simulink model "ASM_Traffic_new"  (R2024a)
settings: Solver=ode1  StartTime=SIM.tstart.v  StopTime=SIM.tend.v  FixedStep=SIM.StepSize.v  RelTol=1e-3
PostLoadFcn:
  | if any(exist('dsrtsu_mdlpostloadfcn', 'file') ~= 0), dsrtsu_mdlpostloadfcn('Execute', bdroot); end
  | try, asm_mdl_postloadfcn(bdroot, 'UpdateModel', 3600); catch, disp(lasterr); end,
InitFcn:
  | , if any(exist('rtifpga_mdlclblib', 'file') ~= 0), rtifpga_mdlclblib('Init', bdroot); end,
  | , if any(exist('dsmpb_private', 'file') ~= 0), dsmpb_private('dsmpb_mdlclblib', 'Init', bdroot); end,
undefined symbols (not defined in the file): _to_, a0b2, ASM_BrakeHydraulics_DemoSystems, ASM_VehicleDynamics_DemoSystems, b98103fe8ad365046cd0, BrakeCircuit, CPT, Crankshaft, DiscIntNeverNeededParam, dsmsi, FinalDriveAssembly, MDL, ModeSignals, Pos_BrakePedal_Maneuver, rad, RefSignals, s_to_rpm, SIM, SoftECU, Suspension, Tire, Transmission
libraries: ASM_Traffic_lib x135, simulink x100, ASM_Utils_lib x77, ASM_VehicleDynamics_lib x70, ASM_Environment_lib x22, dsmpblib x20, dsmsilib x15, MDLD_Utils_lib x10, ASM_BrakeHydraulics_lib x3
(part 30 of 63)

== system ASM_Traffic_new/VehicleDynamics/Interface_Out/Plant_ModelSignals/Sw_r_Tire[1:intern;2:extern]_ ==
  In1 : Inport
  Gain : Gain  SaturateOnIntegerOverflow=on  OutDataTypeStr=Inherit: Same as input  ParamDataTypeStr=Inherit: Same as input
  Out1 : Outport  VectorParamsAs1DForOutWhenUnconnected=off
  wires:
  In1/1 -> Gain/1
  Gain/1 -> Out1/1

== system ASM_Traffic_new/VehicleDynamics/Interface_Out/Plant_ModelSignals/Trq_Max_Brake[Nm]_ ==
  In1 : Inport
  Gain : Gain  SaturateOnIntegerOverflow=on  OutDataTypeStr=Inherit: Same as input  ParamDataTypeStr=Inherit: Same as input
  Out1 : Outport  VectorParamsAs1DForOutWhenUnconnected=off
  wires:
  Gain/1 -> Out1/1
  In1/1 -> Gain/1

== system ASM_Traffic_new/VehicleDynamics/Interface_Out/Plant_ModelSignals/Trq_SteeringWheel[Nm]_ ==
  In1 : Inport
  Gain : Gain  SaturateOnIntegerOverflow=on  OutDataTypeStr=Inherit: Same as input  ParamDataTypeStr=Inherit: Same as input
  Out1 : Outport  VectorParamsAs1DForOutWhenUnconnected=off
  wires:
  Gain/1 -> Out1/1
  In1/1 -> Gain/1

== system ASM_Traffic_new/VehicleDynamics/Interface_Out/Plant_ModelSignals/YawRate_Vehicle_CoG[deg|s]_ ==
  In1 : Inport
  Gain : Gain  SaturateOnIntegerOverflow=on  OutDataTypeStr=Inherit: Same as input  ParamDataTypeStr=Inherit: Same as input
  Out1 : Outport  VectorParamsAs1DForOutWhenUnconnected=off
  wires:
  Gain/1 -> Out1/1
  In1/1 -> Gain/1

== system ASM_Traffic_new/VehicleDynamics/Interface_Out/Plant_ModelSignals/a_Vehicle[x;y;z][m|s2]_ ==
  In1 : Inport
  Gain : Gain  SaturateOnIntegerOverflow=on  OutDataTypeStr=Inherit: Same as input  ParamDataTypeStr=Inherit: Same as input
  Out1 : Outport  VectorParamsAs1DForOutWhenUnconnected=off
  wires:
  In1/1 -> Gain/1
  Gain/1 -> Out1/1

== system ASM_Traffic_new/VehicleDynamics/Interface_Out/Plant_ModelSignals/a_x_Vehicle_CoG[m|s2]_ ==
  In1 : Inport
  Gain : Gain  SaturateOnIntegerOverflow=on  OutDataTypeStr=Inherit: Same as input  ParamDataTypeStr=Inherit: Same as input
  Out1 : Outport  VectorParamsAs1DForOutWhenUnconnected=off
  wires:
  Gain/1 -> Out1/1
  In1/1 -> Gain/1

== system ASM_Traffic_new/VehicleDynamics/Interface_Out/Plant_ModelSignals/a_y_Vehicle_CoG[m|s2]_ ==
  In1 : Inport
  Gain : Gain  SaturateOnIntegerOverflow=on  OutDataTypeStr=Inherit: Same as input  ParamDataTypeStr=Inherit: Same as input
  Out1 : Outport  VectorParamsAs1DForOutWhenUnconnected=off
  wires:
  Gain/1 -> Out1/1
  In1/1 -> Gain/1

== system ASM_Traffic_new/VehicleDynamics/Interface_Out/Plant_ModelSignals/a_z_Vehicle_CoG[m|s2]_ ==
  In1 : Inport
  Gain : Gain  SaturateOnIntegerOverflow=on  OutDataTypeStr=Inherit: Same as input  ParamDataTypeStr=Inherit: Same as input
  Out1 : Outport  VectorParamsAs1DForOutWhenUnconnected=off
  wires:
  Gain/1 -> Out1/1
  In1/1 -> Gain/1

== system ASM_Traffic_new/VehicleDynamics/Interface_Out/Plant_ModelSignals/i_Steering_Mean[]_ ==
  In1 : Inport
  Gain : Gain  SaturateOnIntegerOverflow=on  OutDataTypeStr=Inherit: Same as input  ParamDataTypeStr=Inherit: Same as input
  Out1 : Outport  VectorParamsAs1DForOutWhenUnconnected=off
  wires:
  Gain/1 -> Out1/1
  In1/1 -> Gain/1

== system ASM_Traffic_new/VehicleDynamics/Interface_Out/Plant_ModelSignals/m_TotalVehicle[kg]_ ==
  In1 : Inport
  Gain : Gain  SaturateOnIntegerOverflow=on  OutDataTypeStr=Inherit: Same as input  ParamDataTypeStr=Inherit: Same as input
  Out1 : Outport  VectorParamsAs1DForOutWhenUnconnected=off
  wires:
  Gain/1 -> Out1/1
  In1/1 -> Gain/1

== system ASM_Traffic_new/VehicleDynamics/Interface_Out/Plant_ModelSignals/omega_Mean_Wheel[rad|s]_ ==
  In1 : Inport
  Gain : Gain  SaturateOnIntegerOverflow=on  OutDataTypeStr=Inherit: Same as input  ParamDataTypeStr=Inherit: Same as input
  Out1 : Outport  VectorParamsAs1DForOutWhenUnconnected=off
  wires:
  Gain/1 -> Out1/1
  In1/1 -> Gain/1

== system ASM_Traffic_new/VehicleDynamics/Interface_Out/Plant_ModelSignals/omega_Wheel[FL;FR;RL;RR][rad|s]_ ==
  In1 : Inport
  Gain : Gain  SaturateOnIntegerOverflow=on  OutDataTypeStr=Inherit: Same as input  ParamDataTypeStr=Inherit: Same as input
  Out1 : Outport  VectorParamsAs1DForOutWhenUnconnected=off
  wires:
  Gain/1 -> Out1/1
  In1/1 -> Gain/1

== system ASM_Traffic_new/VehicleDynamics/Interface_Out/Plant_ModelSignals/omega_Wheel[rad|s]_ ==
  In1 : Inport
  Gain : Gain  SaturateOnIntegerOverflow=on  OutDataTypeStr=Inherit: Same as input  ParamDataTypeStr=Inherit: Same as input
  Out1 : Outport  VectorParamsAs1DForOutWhenUnconnected=off
  wires:
  Gain/1 -> Out1/1
  In1/1 -> Gain/1

== system ASM_Traffic_new/VehicleDynamics/Interface_Out/Plant_ModelSignals/r_Dyn_Tire[FL;FR;RL;RR][m]_ ==
  In1 : Inport
  Gain : Gain  SaturateOnIntegerOverflow=on  OutDataTypeStr=Inherit: Same as input  ParamDataTypeStr=Inherit: Same as input
  Out1 : Outport  VectorParamsAs1DForOutWhenUnconnected=off
  wires:
  Gain/1 -> Out1/1
  In1/1 -> Gain/1

== system ASM_Traffic_new/VehicleDynamics/Interface_Out/Plant_ModelSignals/r_Tire_extern[m]_ ==
  In1 : Inport
  Gain : Gain  SaturateOnIntegerOverflow=on  OutDataTypeStr=Inherit: Same as input  ParamDataTypeStr=Inherit: Same as input
  Out1 : Outport  VectorParamsAs1DForOutWhenUnconnected=off
  wires:
  In1/1 -> Gain/1
  Gain/1 -> Out1/1

== system ASM_Traffic_new/VehicleDynamics/Interface_Out/Plant_ModelSignals/s_Vehicle[m]_ ==
  In1 : Inport
  Gain : Gain  SaturateOnIntegerOverflow=on  OutDataTypeStr=Inherit: Same as input  ParamDataTypeStr=Inherit: Same as input
  Out1 : Outport  VectorParamsAs1DForOutWhenUnconnected=off
  wires:
  Gain/1 -> Out1/1
  In1/1 -> Gain/1

== system ASM_Traffic_new/VehicleDynamics/Interface_Out/Plant_ModelSignals/v_Vehicle[km|h]_ ==
  In1 : Inport
  Gain : Gain  SaturateOnIntegerOverflow=on  OutDataTypeStr=Inherit: Same as input  ParamDataTypeStr=Inherit: Same as input
  Out1 : Outport  VectorParamsAs1DForOutWhenUnconnected=off
  wires:
  Gain/1 -> Out1/1
  In1/1 -> Gain/1

== system ASM_Traffic_new/VehicleDynamics/Interface_Out/Plant_ModelSignals/v_Vehicle[x;y;z][km|h]_ ==
  In1 : Inport
  Gain : Gain  SaturateOnIntegerOverflow=on  OutDataTypeStr=Inherit: Same as input  ParamDataTypeStr=Inherit: Same as input
  Out1 : Outport  VectorParamsAs1DForOutWhenUnconnected=off
  wires:
  Gain/1 -> Out1/1
  In1/1 -> Gain/1

== system ASM_Traffic_new/VehicleDynamics/Interface_Out/Plant_ModelSignals/v_Vehicle_dt[x;y;z][m|s2]_ ==
  In1 : Inport
  Gain : Gain  SaturateOnIntegerOverflow=on  OutDataTypeStr=Inherit: Same as input  ParamDataTypeStr=Inherit: Same as input
  Out1 : Outport  VectorParamsAs1DForOutWhenUnconnected=off
  wires:
  Gain/1 -> Out1/1
  In1/1 -> Gain/1

== system ASM_Traffic_new/VehicleDynamics/Interface_Out/Plant_ModelSignals/v_x_Vehicle_CoG[km|h]_ ==
  In1 : Inport
  Gain : Gain  SaturateOnIntegerOverflow=on  OutDataTypeStr=Inherit: Same as input  ParamDataTypeStr=Inherit: Same as input
  Out1 : Outport  VectorParamsAs1DForOutWhenUnconnected=off
  wires:
  Gain/1 -> Out1/1
  In1/1 -> Gain/1

== system ASM_Traffic_new/VehicleDynamics/Interface_Out/Plant_ModelSignals/v_y_Vehicle_CoG[km|h]_ ==
  In1 : Inport
  Gain : Gain  SaturateOnIntegerOverflow=on  OutDataTypeStr=Inherit: Same as input  ParamDataTypeStr=Inherit: Same as input
  Out1 : Outport  VectorParamsAs1DForOutWhenUnconnected=off
  wires:
  Gain/1 -> Out1/1
  In1/1 -> Gain/1

== system ASM_Traffic_new/VehicleDynamics/Interface_Out/Plant_ModelSignals/v_z_Vehicle_CoG[km|h]_ ==
  In1 : Inport
  Gain : Gain  SaturateOnIntegerOverflow=on  OutDataTypeStr=Inherit: Same as input  ParamDataTypeStr=Inherit: Same as input
  Out1 : Outport  VectorParamsAs1DForOutWhenUnconnected=off
  wires:
  Gain/1 -> Out1/1
  In1/1 -> Gain/1

== system ASM_Traffic_new/VehicleDynamics/Interface_Out/Plant_ModelSignals/w_Vehicle[x;y;z][deg|s]_ ==
  In1 : Inport
  Gain : Gain  SaturateOnIntegerOverflow=on  OutDataTypeStr=Inherit: Same as input  ParamDataTypeStr=Inherit: Same as input
  Out1 : Outport  VectorParamsAs1DForOutWhenUnconnected=off
  wires:
  Gain/1 -> Out1/1
  In1/1 -> Gain/1

== system ASM_Traffic_new/VehicleDynamics/Interface_Out/Plant_ModelSignals/w_Vehicle_dt[x;y;z][rad|s2]_ ==
  In1 : Inport
  Gain : Gain  SaturateOnIntegerOverflow=on  OutDataTypeStr=Inherit: Same as input  ParamDataTypeStr=Inherit: Same as input
  Out1 : Outport  VectorParamsAs1DForOutWhenUnconnected=off
  wires:
  Gain/1 -> Out1/1
  In1/1 -> Gain/1

== system ASM_Traffic_new/VehicleDynamics/Interface_Out/Plant_ModelSignals/w_x_Vehicle_CoG[rad|s2]_ ==
  In1 : Inport
  Gain : Gain  SaturateOnIntegerOverflow=on  OutDataTypeStr=Inherit: Same as input  ParamDataTypeStr=Inherit: Same as input
  Out1 : Outport  VectorParamsAs1DForOutWhenUnconnected=off
  wires:
  Gain/1 -> Out1/1
  In1/1 -> Gain/1

== system ASM_Traffic_new/VehicleDynamics/Interface_Out/Plant_ModelSignals/w_y_Vehicle_CoG[rad|s2]_ ==
  In1 : Inport
  Gain : Gain  SaturateOnIntegerOverflow=on  OutDataTypeStr=Inherit: Same as input  ParamDataTypeStr=Inherit: Same as input
  Out1 : Outport  VectorParamsAs1DForOutWhenUnconnected=off
  wires:
  In1/1 -> Gain/1
  Gain/1 -> Out1/1

== system ASM_Traffic_new/VehicleDynamics/Interface_Out/Plant_ModelSignals/w_z_Vehicle_CoG[rad|s2]_ ==
  In1 : Inport
  Gain : Gain  SaturateOnIntegerOverflow=on  OutDataTypeStr=Inherit: Same as input  ParamDataTypeStr=Inherit: Same as input
  Out1 : Outport  VectorParamsAs1DForOutWhenUnconnected=off
  wires:
  Gain/1 -> Out1/1
  In1/1 -> Gain/1

== system ASM_Traffic_new/VehicleDynamics/Plant/Sw_Plant_Signals/Angle_Gamma_FL_Wheel[deg] ==
  SoftECU : Inport
  RealECU : Inport  Port=2
  Const_Angle_Gamma_FL_Wheel[deg] : Constant  Value=0
  MultiPortSwitch : MultiPortSwitch
  Sw_Angle_Gamma_FL_Wheel[1SoftECU|2RealECU|3Const] : Constant  Value=CPT.MDL_SW.Sw_Angle_Gamma_FL_Wheel.v
  Angle_Gamma_FL_Wheel[deg] : Outport  VectorParamsAs1DForOutWhenUnconnected=off
  wires:
  MultiPortSwitch/1 -> Angle_Gamma_FL_Wheel[deg]/1
  Const_Angle_Gamma_FL_Wheel[deg]/1 -> MultiPortSwitch/4
  RealECU/1 -> MultiPortSwitch/3
  SoftECU/1 -> MultiPortSwitch/2
  Sw_Angle_Gamma_FL_Wheel[1SoftECU|2RealECU|3Const]/1 -> MultiPortSwitch/1

== system ASM_Traffic_new/VehicleDynamics/Plant/Sw_Plant_Signals/Displ_SteeringRod[Displ;Displ_dt][m;m|s] ==
  SoftECU : Inport
  RealECU : Inport  Port=2
  Const_Displ_SteeringRod[Displ;Displ_dt][m;m|s] : Constant  Value=[0;0]
  MultiPortSwitch : MultiPortSwitch
  Sw_Displ_SteeringRod[1SoftECU|2RealECU|3Const] : Constant  Value=CPT.MDL_SW.Sw_Displ_SteeringRod.v
  Displ_SteeringRod[Displ;Displ_dt][m;m|s] : Outport  VectorParamsAs1DForOutWhenUnconnected=off
  wires:
  MultiPortSwitch/1 -> Displ_SteeringRod[Displ;Displ_dt][m;m|s]/1
  Const_Displ_SteeringRod[Displ;Displ_dt][m;m|s]/1 -> MultiPortSwitch/4
  RealECU/1 -> MultiPortSwitch/3
  SoftECU/1 -> MultiPortSwitch/2
  Sw_Displ_SteeringRod[1SoftECU|2RealECU|3Const]/1 -> MultiPortSwitch/1

== system ASM_Traffic_new/VehicleDynamics/Plant/Sw_Plant_Signals/EPSMotorStates_External[Angle;Angle_dt][rad;rad|s] ==
  SoftECU : Inport
  RealECU : Inport  Port=2
  Const_EPSMotorStates_External[Angle;Angle_dt][rad;rad|s] : Constant  Value=[0;0]
  MultiPortSwitch : MultiPortSwitch
  Sw_EPSMotorStates_External[1SoftECU|2RealECU|3Const] : Constant  Value=CPT.MDL_SW.Sw_EPSMotorStates_External.v
  EPSMotorStates_External[Angle;Angle_dt][rad;rad|s] : Outport  VectorParamsAs1DForOutWhenUnconnected=off
  wires:
  Sw_EPSMotorStates_External[1SoftECU|2RealECU|3Const]/1 -> MultiPortSwitch/1
  SoftECU/1 -> MultiPortSwitch/2
  RealECU/1 -> MultiPortSwitch/3
  Const_EPSMotorStates_External[Angle;Angle_dt][rad;rad|s]/1 -> MultiPortSwitch/4
  MultiPortSwitch/1 -> EPSMotorStates_External[Angle;Angle_dt][rad;rad|s]/1

== system ASM_Traffic_new/VehicleDynamics/Plant/Sw_Plant_Signals/omega_Wheel[FL;FR;RL;RR][rad|s] ==
  SoftECU : Inport
  RealECU : Inport  Port=2
  Const_omega_Wheel[FL;FR;RL;RR][rad|s] : Constant  Value=[0 0 0 0]
  MultiPortSwitch : MultiPortSwitch
  Sw_omega_Wheel[1SoftECU|2RealECU|3Const] : Constant  Value=CPT.MDL_SW.Sw_omega_Wheel.v
  omega_Wheel[FL;FR;RL;RR][rad|s] : Outport  VectorParamsAs1DForOutWhenUnconnected=off
  wires:
  Sw_omega_Wheel[1SoftECU|2RealECU|3Const]/1 -> MultiPortSwitch/1
  SoftECU/1 -> MultiPortSwitch/2
  RealECU/1 -> MultiPortSwitch/3
  MultiPortSwitch/1 -> omega_Wheel[FL;FR;RL;RR][rad|s]/1
  Const_omega_Wheel[FL;FR;RL;RR][rad|s]/1 -> MultiPortSwitch/4

== system ASM_Traffic_new/VehicleDynamics/Plant/UserInterface/ASMSignalBus_Plant ==
  In : Inport
  Terminator_1 : Terminator
  tag scope: ASMBUS_VehicleDynamics_Plant=global
  wires:
  In/1 -> [ASMBUS_VehicleDynamics_Plant]  "Plant"
  [ASMBUS_VehicleDynamics_Plant] -> Terminator_1/1

== system ASM_Traffic_new/VehicleDynamics/Plant/UserInterface/DISP_Plant ==
  In : Inport
  Accelerations : Subsystem
  Aerodynamics : Subsystem
  Brake : Subsystem
  Bus Selector2 : BusSelector  OutputSignals=Suspension,VehicleMovement.Positions,VehicleMovement.Velocities,VehicleMovement.Accelerations,Wheel,Tire,Aerodynamics,Steering,Brake,VehicleMovement.SensorMotion.Sensor1
  Overview : Subsystem
  Positions : Subsystem
  Sensor1 : Subsystem
  Steering : Subsystem
  Suspension : Subsystem
  Tire : Subsystem
  Velocities : Subsystem
  WheelSpeeds : Subsystem
  wires:
  Bus Selector2/10 -> Sensor1/1(Sensor1)  "<Sensor1>"
  Bus Selector2/5 -> WheelSpeeds/1(WheelSpeeds)  "<Wheel>"
  Bus Selector2/4 -> Accelerations/1(Accelerations), Overview/2(Accelerations)  "<Accelerations>"
  In/1 -> Bus Selector2/1
  Bus Selector2/8 -> Steering/1(Steering)  "<Steering>"
  Bus Selector2/3 -> Velocities/1(Velocities), Overview/1(Velocities)  "<Velocities>"
  Bus Selector2/6 -> Tire/1(Tire)  "<Tire>"
  Bus Selector2/7 -> Aerodynamics/1(Aerodynamics)  "<Aerodynamics>"
  Bus Selector2/9 -> Brake/1(Brake)  "<Brake>"
  Bus Selector2/2 -> Positions/1(Positions)  "<Positions>"
  Bus Selector2/1 -> Suspension/1(Suspension)  "<Suspension>"

== system ASM_Traffic_new/VehicleDynamics/Plant/UserInterface/PAR_Plant ==
  BrakeHydraulics_DistributionPattern_Switch : Subsystem
      mask Display: disp('BrakeHydraulics_DistributionPattern_Switch')
  Bus Creator : BusCreator  Inputs=3
  Bus Creator1 : BusCreator  Inputs=1
  Bus Creator2 : BusCreator  Inputs=1
  Bus Creator3 : BusCreator  Inputs=2
  ModelDesk_MC_ID_VehicleDynamics : ASM_Utils_lib/ModelDeskInterface/ModelDesk_MC  Tag=ASM_MAINCOMPONENT  Editable=off  MainComponent=VehicleDynamics
  ROTATION_SWITCH : ASM_VehicleDynamics_lib/VehicleDynamics/Suspension/Common/ROTATION_SWITCH  Tag=ASM_SUBCOMPONENT  Sw_Rotation=MDL.VehicleDynamics.SW_Rotation  ASMProperties=struct('Name','ROTATION_SWITCH','Version','2.0','Library','ASM_VehicleDynamics_lib')  ASMInstanceName=rotation_switch  ASMInstanceID=1
  Suspension_Inits : Subsystem
      mask Display: disp('Suspension Inits')
  Tire_Switches : Subsystem
      mask Display: disp('Tire Switches')
  Out : Outport  VectorParamsAs1DForOutWhenUnconnected=off
  wires:
  ROTATION_SWITCH/1 -> Bus Creator3/2  "Sw_Rotation[1Cardan|2ToeCamberCaster]"
  Bus Creator3/1 -> Bus Creator/3  "Suspension"
  Bus Creator/1 -> Out/1  "UserInterface"
  Bus Creator2/1 -> Bus Creator/2  "BrakeHydraulics"
  Tire_Switches/1(Tire_Switches) -> Bus Creator1/1  "Tire"
  Suspension_Inits/1(Suspension_Init) -> Bus Creator3/1
  BrakeHydraulics_DistributionPattern_Switch/1(Sw_DistributionPattern_[1X|2II]) -> Bus Creator2/1
  Bus Creator1/1 -> Bus Creator/1  "Tire"

== system ASM_Traffic_new/VehicleDynamics/Plant/VehicleDynamics/ASMSignalCollector ==
  Bus Selector : BusSelector  OutputSignals=Coef_RollingRes_Mean[]
  Bus Selector1 : BusSelector  OutputSignals=Forces.F_x_Aero_CoorSys_V[N]
  Bus Selector2 : BusSelector  OutputSignals=MassForcesAndTorques.GravitationalForces.F_Vehicle_Gravitational[x;y;z][N]
  BusCreator : BusCreator  Inputs=9
  Driving_Resistances : Subsystem
  ASMSignalBus : Outport  VectorParamsAs1DForOutWhenUnconnected=off
  wires:
  [ASMBUS_VehicleDynamics_WheelSpeed] -> BusCreator/4
  [ASMBUS_VehicleDynamics_Aerodynamics] -> Bus Selector1/1, BusCreator/3
  [ASMBUS_VehicleDynamics_Brake] -> BusCreator/6
  Driving_Resistances/1(F_Driving_Res[N]) -> BusCreator/9
  Bus Selector2/1 -> Driving_Resistances/1(F_Vehicle_Gravitational[x;y;z][N])  "<F_Vehicle_Gravitational[x;y;z][N]>"
  Bus Selector/1 -> Driving_Resistances/2(Coef_RollingRes_Mean[])  "<Coef_RollingRes_Mean[]>"
  [ASMBUS_VehicleDynamics_Steering] -> BusCreator/5
  [ASMBUS_VehicleDynamics_VehicleMovement] -> Bus Selector2/1, BusCreator/1
  Bus Selector1/1 -> Driving_Resistances/3(F_x_Aero_CoorSys_V[N])  "<F_x_Aero_CoorSys_V[N]>"
  [ASMBUS_VehicleDynamics_Suspension] -> BusCreator/7
  [ASMBUS_VehicleDynamics_Tire] -> Bus Selector/1, BusCreator/2
  BusCreator/1 -> ASMSignalBus/1  "VehicleDynamics"
  [ASMBUS_VehicleDynamics_Steering_Rod_Back_Calc] -> BusCreator/8

== system ASM_Traffic_new/VehicleDynamics/Plant/VehicleDynamics/Brake ==
  Reset[] : Inport
  Pos_BrakePedal[%] : Inport  Port=2
  IO_Signals : Inport  Port=3
  p_Ambient[Pa] : Inport  Port=4
  Sw_ParkingBrake[0Off|1On] : Inport  Port=5
  T_Ambient[degC] : Inport  Port=6
  Pos_AccPedal[%] : Inport  Port=7
  Sw_DistributionPattern[1X|2II] : Inport  Port=8
  ASMSignalCollector : Subsystem
  BRAKE_DISC : ASM_VehicleDynamics_lib/VehicleDynamics/Brake/BRAKE_DISC  Tag=ASM_SUBCOMPONENT  Const_Fric_Coef_FL=MDL.VehicleDynamics.BrakeDisc.FL.Const_Coef_Fric  Const_Fric_Coef_FR=MDL.VehicleDynamics.BrakeDisc.FR.Const_Coef_Fric  Const_Fric_Coef_RL=MDL.VehicleDynamics.BrakeDisc.RL.Const_Coef_Fric  Const_Fric_Coef_RR=MDL.VehicleDynamics.BrakeDisc.RR.Const_Coef_Fric  Const_A_FL=MDL.VehicleDynamics.BrakeDisc.FL.Const_A_Fric  Const_A_FR=MDL.VehicleDynamics.BrakeDisc.FR.Const_A_Fric  Const_A_RL=MDL.VehicleDynamics.BrakeDisc.RL.Const_A_Fric  Const_A_RR=MDL.VehicleDynamics.BrakeDisc.RR.Const_A_Fric  Const_r_FL=MDL.VehicleDynamics.BrakeDisc.FL.Const_r  Const_r_FR=MDL.VehicleDynamics.BrakeDisc.FR.Const_r  Const_r_RL=MDL.VehicleDynamics.BrakeDisc.RL.Const_r  Const_r_RR=MDL.VehicleDynamics.BrakeDisc.RR.Const_r  ASMProperties=struct('Name','BRAKE_DISC','Version','5.0','Library','ASM_VehicleDynamics_lib')  ASMInstanceName=brake_disc  ASMInstanceID=1
  BRAKE_HYDRAULICS : Subsystem  Tag=BrakeHydraulics_BrakeCircuit
  Bus Selector : BusSelector  OutputSignals=Ctrl_HydPump[0_1],Ctrl_PreChargeValve_1[0_1],Ctrl_PreChargeValve_2[0_1],Ctrl_ChangeOverValve_1[0_1],Ctrl_ChangeOverValve_2[0_1],Ctrl_InletValve_FL[0_1],Ctrl_InletValve_FR[0_1],Ctrl_InletValve_RL[0_1],Ctrl_InletValve_RR[0_1],Ctrl_OutletValve_FL[0_1],Ctrl_OutletValve_FR[0_1],Ctrl_OutletValve_RL[0_1],Ctrl_OutletValve_RR[0_1],ECU_ESP_Mode[0None|1ABS|2ESP|3ASR]
  Bus Selector1 : BusSelector  OutputSignals=Enable_p_Brake_Desired[0|1],p_Brake_Desired[bar]
  Constant : Constant  Value=0
  ForceParkingBrake : Subsystem
  Goto Tag Visibility : GotoTagVisibility  GotoTag=TAG_DISP_BrkHyd_MasterBrakeCylinder
  Goto Tag Visibility1 : GotoTagVisibility  GotoTag=ASMBUS_VehicleDynamics_VacuumServo
  Goto Tag Visibility2 : GotoTagVisibility  GotoTag=ASMBUS_VehicleDynamics_Manifold
  Goto Tag Visibility3 : GotoTagVisibility  GotoTag=ASMBUS_VehicleDynamics_BrakeHydraulics
  Goto Tag Visibility4 : GotoTagVisibility  GotoTag=ASMBUS_VehicleDynamics_BrakeDisc
  MANIFOLD_PRESSURE : ASM_VehicleDynamics_lib/VehicleDynamics/Brake/MANIFOLD_PRESSURE  Tag=ASM_SUBCOMPONENT  Map_p_Man=MDL.VehicleDynamics.ManifoldPressure.Map_p_Man  ASMProperties=struct('Name','MANIFOLD_PRESSURE','Version','2.0','Library','ASM_VehicleDynamics_lib')  ASMInstanceName=manifold_pressure  ASMInstanceID=1
  MASTER_BRAKE_CYLINDER : ASM_BrakeHydraulics_lib/BrakeHydraulics/BrakeCylinders/MASTER_BRAKE_CYLINDER  Tag=ASM_SUBCOMPONENT  Const_p_max=MDL.BrkHyd.MasterBrakeCylinderLinear.Const_p_max  Map_BrakeForce=MDL.BrkHyd.MasterBrakeCylinder.Map_BrakeForce  Const_r_piston=MDL.BrkHyd.MasterBrakeCylinder.Const_r_piston  Const_displ_max_piston=MDL.BrkHyd.MasterBrakeCylinder.Const_displ_max_piston  SW_MasterBrakeCylinder_Mode=MDL.BrkHyd.SW_MasterBrakeCylinderType.v  ASMProperties=struct('Name','MASTER_BRAKE_CYLINDER','Version','8.0','Library','ASM_BrakeHydraulics_lib')  ASMInstanceName=master_brake_cylinder  ASMInstanceID=1
  OpenBrakeCircuit : ASM_Utils_lib/Miscellaneous/OpenSystem  popupLibBlk=<select here>  popupTargetDemo=<select here>  Demosystem=BrakeHydraulics_BrakeCircuit  variantLib=ASM_BrakeHydraulics_DemoSystems/BrakeCircuit
  UnitConversion : ASM_Utils_lib/UnitConversion/UnitConversion  Selection=Pa_to_bar
  VACUUM_SERVO : ASM_VehicleDynamics_lib/VehicleDynamics/Brake/VACUUM_SERVO  Tag=ASM_SUBCOMPONENT  Const_F_OutputPoint=MDL.VehicleDynamics.VacuumServo.Const_F_OutputPoint  Const_p_OutputPoint=MDL.VehicleDynamics.VacuumServo.Const_p_OutputPoint  Const_F_Max_PistonRod=MDL.VehicleDynamics.VacuumServo.Const_F_Max_PistonRod  Const_p_nom_VaccumChamber=MDL.VehicleDynamics.VacuumServo.Const_p_nom_VaccumChamber  Const_V_VacuumChamber=MDL.VehicleDynamics.VacuumServo.Const_V_VacuumChamber  Const_V_RearChamber=MDL.VehicleDynamics.VacuumServo.Const_V_RearChamber  Const_A_Connect_BellValve=MDL.VehicleDynamics.VacuumServo.Const_A_Connect_BellValve  Const_A_Boost_BellValve=MDL.VehicleDynamics.VacuumServo.Const_A_Boost_BellValve  Const_A_MainfoldValve=MDL.VehicleDynamics.VacuumServo.Const_A_MainfoldValve  Const_A_Leakage_MainfoldValve=MDL.VehicleDynamics.VacuumServo.Const_A_Leakage_MainfoldValve  Const_c_spring=MDL.VehicleDynamics.VacuumServo.Const_c_spring  StepSize=SIM.StepSize  ASMProperties=struct('Name','VACUUM_SERVO','Version','4.0','Library','ASM_VehicleDynamics_lib')  ASMInstanceName=vacuum_servo  ASMInstanceID=1
  avoid_incomplete_trace2source : Subsystem
  avoid_incomplete_trace2source1 : Subsystem
  avoid_incomplete_trace2source2 : Subsystem
  ASMSignalBus : Outport  VectorParamsAs1DForOutWhenUnconnected=off
  Trq_Brake[FL,FR,RL,RR][Nm] : Outport  Port=2  VectorParamsAs1DForOutWhenUnconnected=off
  tag scope: ASMBUS_VehicleDynamics_BrakeDisc=scoped, ASMBUS_VehicleDynamics_BrakeHydraulics=scoped, ASMBUS_VehicleDynamics_Manifold=scoped, ASMBUS_VehicleDynamics_VacuumServo=scoped, TAG_DISP_BrkHyd_MasterBrakeCylinder=scoped
  wires:
  avoid_incomplete_trace2source2/1(Out1) -> MASTER_BRAKE_CYLINDER/5
  avoid_incomplete_trace2source1/1(Out1) -> MASTER_BRAKE_CYLINDER/4
  Bus Selector1/2 -> avoid_incomplete_trace2source2/1(In1)  "<p_Brake_Desired[bar]>"
  Bus Selector1/1 -> avoid_incomplete_trace2source1/1(In1)  "<Enable_p_Brake_Desired[0|1]>"
  avoid_incomplete_trace2source/1(Out1) -> MANIFOLD_PRESSURE/1
  Pos_AccPedal[%]/1 -> avoid_incomplete_trace2source/1(In1)
  MASTER_BRAKE_CYLINDER/1 -> [TAG_DISP_BrkHyd_MasterBrakeCylinder]
  VACUUM_SERVO/2 -> MASTER_BRAKE_CYLINDER/3
  MASTER_BRAKE_CYLINDER/2 -> BRAKE_DISC/2
  MASTER_BRAKE_CYLINDER/4 -> VACUUM_SERVO/2
  MASTER_BRAKE_CYLINDER/3 -> VACUUM_SERVO/1, BRAKE_HYDRAULICS/1(p_MasterBrakeCylinder[bar])
  Sw_DistributionPattern[1X|2II]/1 -> BRAKE_HYDRAULICS/2(Sw_DistributionPattern[1X|2II])
  Bus Selector/14 -> BRAKE_HYDRAULICS/17(ECU_Mode[0None|1ABS|2ESP|3ASR])  "<ECU_ESP_Mode[0None|1ABS|2ESP|3ASR]>"
  ASMSignalCollector/1(ASMSignalBus) -> ASMSignalBus/1
  BRAKE_DISC/2 -> Trq_Brake[FL,FR,RL,RR][Nm]/1
  BRAKE_DISC/1 -> [ASMBUS_VehicleDynamics_BrakeDisc]
  IO_Signals/1 -> Bus Selector1/1, Bus Selector/1
  BRAKE_HYDRAULICS/1(ASMSignalBus) -> [ASMBUS_VehicleDynamics_BrakeHydraulics]
  Reset[]/1 -> BRAKE_HYDRAULICS/3(Reset[]), VACUUM_SERVO/9
  Pos_BrakePedal[%]/1 -> MASTER_BRAKE_CYLINDER/1, VACUUM_SERVO/8
  Bus Selector/1 -> BRAKE_HYDRAULICS/4(Ctrl_HydPump[0_1])  "<Ctrl_HydPump[0_1]>"
  Bus Selector/2 -> BRAKE_HYDRAULICS/5(Ctrl_PreChargeValve_1[])  "<Ctrl_PreChargeValve_1[0_1]>"
  Bus Selector/3 -> BRAKE_HYDRAULICS/6(Ctrl_PreChargeValve_2[])  "<Ctrl_PreChargeValve_2[0_1]>"
  Bus Selector/4 -> BRAKE_HYDRAULICS/7(Ctrl_ChangeOverValve_1[])  "<Ctrl_ChangeOverValve_1[0_1]>"
  Bus Selector/5 -> BRAKE_HYDRAULICS/8(Ctrl_ChangeOverValve_2[])  "<Ctrl_ChangeOverValve_2[0_1]>"
  Bus Selector/6 -> BRAKE_HYDRAULICS/9(Ctrl_InletValve_FL[])  "<Ctrl_InletValve_FL[0_1]>"
  Bus Selector/7 -> BRAKE_HYDRAULICS/10(Ctrl_InletValve_FR[])  "<Ctrl_InletValve_FR[0_1]>"
  Bus Selector/8 -> BRAKE_HYDRAULICS/11(Ctrl_InletValve_RL[])  "<Ctrl_InletValve_RL[0_1]>"
  Bus Selector/9 -> BRAKE_HYDRAULICS/12(Ctrl_InletValve_RR[])  "<Ctrl_InletValve_RR[0_1]>"
  Bus Selector/10 -> BRAKE_HYDRAULICS/13(Ctrl_OutletValve_FL[])  "<Ctrl_OutletValve_FL[0_1]>"
  Bus Selector/11 -> BRAKE_HYDRAULICS/14(Ctrl_OutletValve_FR[])  "<Ctrl_OutletValve_FR[0_1]>"
  Bus Selector/12 -> BRAKE_HYDRAULICS/15(Ctrl_OutletValve_RL[])  "<Ctrl_OutletValve_RL[0_1]>"
  Bus Selector/13 -> BRAKE_HYDRAULICS/16(Ctrl_OutletValve_RR[])  "<Ctrl_OutletValve_RR[0_1]>"
  Sw_ParkingBrake[0Off|1On]/1 -> ForceParkingBrake/1(Sw_ParkingBrake[0Off|1On])
  VACUUM_SERVO/1 -> [ASMBUS_VehicleDynamics_VacuumServo]
  MANIFOLD_PRESSURE/1 -> [ASMBUS_VehicleDynamics_Manifold]
  UnitConversion/1 -> MASTER_BRAKE_CYLINDER/2, VACUUM_SERVO/3, BRAKE_DISC/3, BRAKE_HYDRAULICS/18(p_Ambient[bar])
  p_Ambient[Pa]/1 -> UnitConversion/1
  Constant/1 -> VACUUM_SERVO/5
  T_Ambient[degC]/1 -> VACUUM_SERVO/4, VACUUM_SERVO/6
  MANIFOLD_PRESSURE/2 -> VACUUM_SERVO/7
  ForceParkingBrake/1(F_ParkingBrake[FL;FR;RL;RR][N]) -> BRAKE_DISC/4
  BRAKE_HYDRAULICS/2(p_Brake[FL,FR,RL,RR][bar]) -> BRAKE_DISC/1

== system ASM_Traffic_new/VehicleDynamics/Plant/VehicleDynamics/CommonVehicleParameters ==
  Bus Selector : BusSelector  OutputSignals=Front.Const_m_Left_Wheel[kg],Front.Const_m_Right_Wheel[kg],Rear.Const_m_Left_Wheel[kg],Rear.Const_m_Right_Wheel[kg],Front.Const_Inertia_Tensor_Left_Wheel[3x3][kgm2],Front.Const_Inertia_Tensor_Right_Wheel[3x3][kgm2],Rear.Const_Inertia_Tensor_Left_Wheel[3x3][kgm2],Rear.Const_Inertia_Tensor_Right_Wheel[3x3][kgm2],Front.Const_Inertia_y_Left_Wheel[kgm2],Front.Const_Inertia_y_Right_Wheel[kgm2],Rear.Const_Inertia_y_Left_Wheel[kgm2],Rear.Const_Inertia_y_Right_Wheel[kgm2],Front.Const_Coef_DynamicBrakeTrq_Left_Wheel[Nm|(rad|s)],Front.Const_Coef_DynamicBrakeTrq_Right_Wheel[Nm|(rad|s)],Rear.Const_Coef_DynamicBrakeTrq_Left_Wheel[Nm|(rad|s)],Rear.Const_Coef_DynamicBrakeTrq_Right_Wheel[Nm|(rad|s)]
  COMMON_VEHICLE_PARAMETERS : ASM_VehicleDynamics_lib/VehicleDynamics/Common_Parameter/COMMON_VEHICLE_PARAMETERS  Tag=ASM_SUBCOMPONENT  Const_m_FL_Wheel=MDL.VehicleDynamics.Wheel.FL.Const_m  Const_m_FR_Wheel=MDL.VehicleDynamics.Wheel.FR.Const_m  Const_m_RL_Wheel=MDL.VehicleDynamics.Wheel.RL.Const_m  Const_m_RR_Wheel=MDL.VehicleDynamics.Wheel.RR.Const_m  Const_Inertia_Tensor_FL_Wheel=MDL.VehicleDynamics.Wheel.FL.Const_Inertia_Tensor  Const_Inertia_Tensor_FR_Wheel=MDL.VehicleDynamics.Wheel.FR.Const_Inertia_Tensor  Const_Inertia_Tensor_RL_Wheel=MDL.VehicleDynamics.Wheel.RL.Const_Inertia_Tensor  Const_Inertia_Tensor_RR_Wheel=MDL.VehicleDynamics.Wheel.RR.Const_Inertia_Tensor  Const_Inertia_y_FL_Wheel=MDL.VehicleDynamics.Wheel.FL.Const_Inertia_y  Const_Inertia_y_FR_Wheel=MDL.VehicleDynamics.Wheel.FR.Const_Inertia_y  Const_Inertia_y_RL_Wheel=MDL.VehicleDynamics.Wheel.RL.Const_Inertia_y  Const_Inertia_y_RR_Wheel=MDL.VehicleDynamics.Wheel.RR.Const_Inertia_y  Const_Coef_DynamicBrakeTrq_FL=MDL.VehicleDynamics.Wheel.FL.Const_Coef_DynamicBrakeTrq  Const_Coef_DynamicBrakeTrq_FR=MDL.VehicleDynamics.Wheel.FR.Const_Coef_DynamicBrakeTrq  Const_Coef_DynamicBrakeTrq_RL=MDL.VehicleDynamics.Wheel.RL.Const_Coef_DynamicBrakeTrq  Const_Coef_DynamicBrakeTrq_RR=MDL.VehicleDynamics.Wheel.RR.Const_Coef_DynamicBrakeTrq  ASMProperties=struct('Name','COMMON_VEHICLE_PARAMETERS','Version','3.0','Library','ASM_VehicleDynamics_lib')  ASMInstanceName=common_vehicle_parameters  ASMInstanceID=1
  Mux : Mux
  Mux2 : Mux
  Rename1 : Subsystem
      mask Display: disp('')
  Rename2 : Subsystem
      mask Display: disp('')
  Rename3 : Subsystem
      mask Display: disp('')
  Rename4 : Subsystem
      mask Display: disp('')
  Rename5 : Subsystem
      mask Display: disp('')
  Rename6 : Subsystem
      mask Display: disp('')
  Rename7 : Subsystem
      mask Display: disp('')
  Rename8 : Subsystem
      mask Display: disp('')
  tag scope: TAG_VehicleDynamics_Coef_DynamicBrakeTrq=scoped, TAG_VehicleDynamics_Inertia_FL_Wheel=scoped, TAG_VehicleDynamics_Inertia_FR_Wheel=scoped, TAG_VehicleDynamics_Inertia_RL_Wheel=scoped, TAG_VehicleDynamics_Inertia_RR_Wheel=scoped, TAG_VehicleDynamics_Inertia_y_FL_Wheel=scoped, TAG_VehicleDynamics_Inertia_y_FR_Wheel=scoped, TAG_VehicleDynamics_Inertia_y_RL_Wheel=scoped, TAG_VehicleDynamics_Inertia_y_RR_Wheel=scoped, TAG_VehicleDynamics_Inertia_y_Wheel=global, TAG_VehicleDynamics_m_FL_Wheel=scoped, TAG_VehicleDynamics_m_FR_Wheel=scoped, TAG_VehicleDynamics_m_RL_Wheel=scoped, TAG_VehicleDynamics_m_RR_Wheel=scoped
  wires:
  Mux2/1 -> [TAG_VehicleDynamics_Inertia_y_Wheel]
  Rename7/1(Out1) -> Mux2/4
  Rename6/1(Out1) -> Mux2/3
  Rename5/1(Out1) -> Mux2/2
  Rename8/1(Out1) -> Mux2/1
  Rename3/1(Out1) -> Mux/4
  Rename2/1(Out1) -> Mux/3
  Rename1/1(Out1) -> Mux/2
  Rename4/1(Out1) -> Mux/1
  Bus Selector/16 -> Rename3/1(In1)  "<Const_Coef_DynamicBrakeTrq_Right_Wheel[Nm|(rad|s)]>"
  Bus Selector/15 -> Rename2/1(In1)  "<Const_Coef_DynamicBrakeTrq_Left_Wheel[Nm|(rad|s)]>"
  Bus Selector/14 -> Rename1/1(In1)  "<Const_Coef_DynamicBrakeTrq_Right_Wheel[Nm|(rad|s)]>"
  Bus Selector/13 -> Rename4/1(In1)  "<Const_Coef_DynamicBrakeTrq_Left_Wheel[Nm|(rad|s)]>"
  Bus Selector/12 -> Rename7/1(In1), [TAG_VehicleDynamics_Inertia_y_RR_Wheel]  "<Const_Inertia_y_Right_Wheel[kgm2]>"
  Bus Selector/11 -> Rename6/1(In1), [TAG_VehicleDynamics_Inertia_y_RL_Wheel]  "<Const_Inertia_y_Left_Wheel[kgm2]>"
  Bus Selector/10 -> Rename5/1(In1), [TAG_VehicleDynamics_Inertia_y_FR_Wheel]  "<Const_Inertia_y_Right_Wheel[kgm2]>"
  Bus Selector/9 -> Rename8/1(In1), [TAG_VehicleDynamics_Inertia_y_FL_Wheel]  "<Const_Inertia_y_Left_Wheel[kgm2]>"
  Bus Selector/8 -> [TAG_VehicleDynamics_Inertia_RR_Wheel]  "<Const_Inertia_Tensor_Right_Wheel[3x3][kgm2]>"
  Bus Selector/7 -> [TAG_VehicleDynamics_Inertia_RL_Wheel]  "<Const_Inertia_Tensor_Left_Wheel[3x3][kgm2]>"
  Bus Selector/6 -> [TAG_VehicleDynamics_Inertia_FR_Wheel]  "<Const_Inertia_Tensor_Right_Wheel[3x3][kgm2]>"
  Bus Selector/5 -> [TAG_VehicleDynamics_Inertia_FL_Wheel]  "<Const_Inertia_Tensor_Left_Wheel[3x3][kgm2]>"
  Bus Selector/4 -> [TAG_VehicleDynamics_m_RR_Wheel]  "<Const_m_Right_Wheel[kg]>"
  Bus Selector/3 -> [TAG_VehicleDynamics_m_RL_Wheel]  "<Const_m_Left_Wheel[kg]>"
  Bus Selector/2 -> [TAG_VehicleDynamics_m_FR_Wheel]  "<Const_m_Right_Wheel[kg]>"
  Bus Selector/1 -> [TAG_VehicleDynamics_m_FL_Wheel]  "<Const_m_Left_Wheel[kg]>"
  COMMON_VEHICLE_PARAMETERS/1 -> Bus Selector/1
  Mux/1 -> [TAG_VehicleDynamics_Coef_DynamicBrakeTrq]

== system ASM_Traffic_new/VehicleDynamics/Plant/VehicleDynamics/DerivativeAddition ==
  Angle_SteeringWheel_Driver[deg] : Inport
  Discrete Derivative : simulink/Discrete/Discrete Derivative  gainval=1.0  ICPrevScaledInput=0.0  OutMin=[]  OutMax=[]  OutDataType=fixdt(1, 16)  OutScaling=2^-10  DoSatur=off
  Mux : Mux  Inputs=2
  SteeringWheel_Driver[Angle;Angle_dt][deg;deg|s] : Outport  VectorParamsAs1DForOutWhenUnconnected=off
  wires:
  Discrete Derivative/1 -> Mux/2
  Mux/1 -> SteeringWheel_Driver[Angle;Angle_dt][deg;deg|s]/1
  Angle_SteeringWheel_Driver[deg]/1 -> Mux/1, Discrete Derivative/1

== system ASM_Traffic_new/VehicleDynamics/Plant/VehicleDynamics/Exchangeable_Plant_Signals ==
  omega_Wheel[rad|s] : Inport
  ASMInterface_RollerDyno : Subsystem
  ASMInterface_Steering : Subsystem
  Bus Creator6 : BusCreator  Inputs=2
  Bus Selector : BusSelector  OutputSignals=SuspensionFront.SuspensionKinematicsFront.Kinematics_Left.Orientation_Left.Angle_Left_Wheel[Alpha;Beta;Gamma][deg].Angle_Gamma_Left_Wheel[deg]
  Bus Selector1 : BusSelector  OutputSignals=Displ_SteeringRod[m],Displ_SteeringRod_dt[m|s]
  Out : Outport  VectorParamsAs1DForOutWhenUnconnected=off
  wires:
  ASMInterface_Steering/1(Out) -> Bus Creator6/1
  Bus Creator6/1 -> Out/1  "Exchangeable_Plant_Signals"
  omega_Wheel[rad|s]/1 -> ASMInterface_RollerDyno/2(omega_Wheel[rad|s])
  ASMInterface_RollerDyno/1(Out) -> Bus Creator6/2
  [ASMBUS_VehicleDynamics_Suspension] -> Bus Selector/1
  Bus Selector/1 -> ASMInterface_RollerDyno/1(Angle_Gamma_FL_Wheel[deg])  "<Angle_Gamma_Left_Wheel[deg]>"
  [ASMBUS_VehicleDynamics_Steering_Rod_Back_Calc] -> Bus Selector1/1
  Bus Selector1/1 -> ASMInterface_Steering/1(Displ_Steering[m])  "<Displ_SteeringRod[m]>"
  Bus Selector1/2 -> ASMInterface_Steering/2(Displ_Steering_dt[m|s])  "<Displ_SteeringRod_dt[m|s]>"

== system ASM_Traffic_new/VehicleDynamics/Plant/VehicleDynamics/Hitch_Vehicle ==
  Q_Articulated_T[6x1] : Inport
  Trq_Hitch_CoorSys_V[x;y;z][Nm] : Inport  Port=2
  M_Articulated_T[6x6] : Inport  Port=3
  Add : Sum
  Demux : Demux  Outputs=[3 3]
  Selector2 : Selector  NumberOfDimensions=2  IndexOptions=Index vector (dialog),Select all  Indices=[1 2 3],-1  OutputSizes=1
      settings: AttributesFormatString=Row:%<Rows>; Col:%<Columns>
  Selector3 : Selector  NumberOfDimensions=2  IndexOptions=Index vector (dialog),Select all  Indices=[1 2 3]+3,-1  OutputSizes=1
      settings: AttributesFormatString=Row:%<Rows>; Col:%<Columns>
  F_External_CoorSys_V[x;y;z][N] : Outport  VectorParamsAs1DForOutWhenUnconnected=off
  Trq_External_CoorSys_V[x;y;z][Nm] : Outport  Port=2  VectorParamsAs1DForOutWhenUnconnected=off
  Stabilization_F_External[3x6] : Outport  Port=3  VectorParamsAs1DForOutWhenUnconnected=off
  Stabilization_Trq_External[3x6] : Outport  Port=4  VectorParamsAs1DForOutWhenUnconnected=off
  wires:
  Add/1 -> Trq_External_CoorSys_V[x;y;z][Nm]/1
  Trq_Hitch_CoorSys_V[x;y;z][Nm]/1 -> Add/2
  M_Articulated_T[6x6]/1 -> Selector2/1, Selector3/1
  Q_Articulated_T[6x1]/1 -> Demux/1
  Selector3/1 -> Stabilization_Trq_External[3x6]/1
  Selector2/1 -> Stabilization_F_External[3x6]/1
  Demux/2 -> Add/1
  Demux/1 -> F_External_CoorSys_V[x;y;z][N]/1

== system ASM_Traffic_new/VehicleDynamics/Plant/VehicleDynamics/OR ==
  In1 : Inport
  In2 : Inport  Port=2
  Data Type Conversion : DataTypeConversion  OutDataTypeStr=double  SaturateOnIntegerOverflow=off  RndMeth=Floor
  Logical Operator : Logic  Operator=OR  AllPortsSameDT=off
  Out : Outport  VectorParamsAs1DForOutWhenUnconnected=off
  wires:
  Logical Operator/1 -> Data Type Conversion/1
  In1/1 -> Logical Operator/1
  In2/1 -> Logical Operator/2
  Data Type Conversion/1 -> Out/1

== system ASM_Traffic_new/VehicleDynamics/Plant/VehicleDynamics/Suspension ==
  q_Wheel[q1_Front;q2_Front;q1_Rear;q2_Rear][] : Inport  PortDimensions=4
  q_Wheel_dt[q1_Front;q2_Front;q1_Rear;q2_Rear][] : Inport  Port=2  PortDimensions=4
  F_Tire[FL;FR;RL;RR][x;y;z][N] : Inport  Port=3
  Trq_Tire[FL;FR;RL;RR][x;y;z][Nm] : Inport  Port=4
  AirSuspensionSignals_In : Inport  Port=5
  Reset[] : Inport  Port=6
  Sw_Rotation[1Cardan|2ToeCamberCaster] : Inport  Port=7
  Displ_SteeringRod_dt[m|s] : Inport  Port=8  PortDimensions=1
  Displ_SteeringRod[m] : Inport  Port=9  PortDimensions=1
  ASMSignalCollector : Subsystem
  Constant : Constant  Value=0
  Goto Tag Visibility : GotoTagVisibility  GotoTag=ASMBUS_SuspensionFront
  Goto Tag Visibility1 : GotoTagVisibility  GotoTag=ASMBUS_SuspensionRear
  Mux{1,5..7,15} (5 alike) : Mux  Inputs=2
  SuspensionFront : Subsystem
  SuspensionRear : Subsystem
  Terminator : Terminator
  Terminator1 : Terminator
  ASMSignalBus : Outport  VectorParamsAs1DForOutWhenUnconnected=off
  SuspensionKinematicRelations_Front : Outport  Port=2  VectorParamsAs1DForOutWhenUnconnected=off
  SuspensionKinematicRelations_Rear : Outport  Port=3  VectorParamsAs1DForOutWhenUnconnected=off
  gFront_dq_Front_dt[2x2][] : Outport  Port=4  VectorParamsAs1DForOutWhenUnconnected=off
  gRear_dq_Rear_dt[2x2][] : Outport  Port=5  VectorParamsAs1DForOutWhenUnconnected=off
  v_Rel_WheelBody[FL,FR,RL,RR][x;y;z][m|s] : Outport  Port=6  VectorParamsAs1DForOutWhenUnconnected=off
  w_Rel_WheelBody[FL,FR,RL,RR][x;y;z][x;y;z][rad|s] : Outport  Port=7  VectorParamsAs1DForOutWhenUnconnected=off
  Pos_Wheels[FL,FR,RL,RR][x;y;z][m] : Outport  Port=8  VectorParamsAs1DForOutWhenUnconnected=off
  gF_Susp[q1_Front;q2_Front;q1_Rear;q2_Rear][] : Outport  Port=9  VectorParamsAs1DForOutWhenUnconnected=off
  UnitVec_y_Wheel_CoorSys_V[FL,FR,RL,RR][x;y;z] : Outport  Port=10  VectorParamsAs1DForOutWhenUnconnected=off
  AirSuspensionSignals_Out : Outport  Port=11  VectorParamsAs1DForOutWhenUnconnected=off
  tag scope: ASMBUS_SuspensionFront=scoped, ASMBUS_SuspensionRear=scoped
  wires:
  SuspensionFront/9(ASMSignalBus) -> [ASMBUS_SuspensionFront]
  Mux6/1 -> Pos_Wheels[FL,FR,RL,RR][x;y;z][m]/1
  Displ_SteeringRod_dt[m|s]/1 -> SuspensionFront/8(Displ_SteeringRod_dt[m|s])
  Reset[]/1 -> SuspensionRear/6(Reset[]), SuspensionFront/6(Reset[])
  SuspensionRear/4(w_Rel_WheelBody[RL,RR][x;y;z][rad|s]) -> Mux7/2
  SuspensionRear/9(ASMSignalBus) -> [ASMBUS_SuspensionRear]
  Displ_SteeringRod[m]/1 -> SuspensionFront/9(Displ_SteeringRod[m])
  q_Wheel[q1_Front;q2_Front;q1_Rear;q2_Rear][]/1 -> SuspensionRear/2(q_Wheel[q1_Front;q2_Front;q1_Rear;q2_Rear][]), SuspensionFront/2(q_Wheel[q1_Front;q2_Front;q1_Rear;q2_Rear][])
  Sw_Rotation[1Cardan|2ToeCamberCaster]/1 -> SuspensionFront/7(Sw_Rotation[1Cardan|2ToeCamberCaster]), SuspensionRear/7(Sw_Rotation[1Cardan|2ToeCamberCaster])
  SuspensionFront/5(gF_Front_Susp[q1,q2][]) -> Mux1/1
  SuspensionRear/5(gF_Rear_Susp[q1,q2][]) -> Mux1/2
  Mux5/1 -> v_Rel_WheelBody[FL,FR,RL,RR][x;y;z][m|s]/1
  SuspensionRear/8(AirSuspensionSignals_Rear) -> Terminator1/1
  SuspensionFront/6(gFront_dq_Front_dt[2x2][]) -> gFront_dq_Front_dt[2x2][]/1
  SuspensionFront/4(w_Rel_WheelBody[FL,FR][x;y;z][rad|s]) -> Mux7/1
  SuspensionRear/6(gRear_dq_Rear_dt[2x2][]) -> gRear_dq_Rear_dt[2x2][]/1
  Constant/1 -> AirSuspensionSignals_Out/1
  SuspensionFront/7(SuspensionKinematicRelations_Front) -> SuspensionKinematicRelations_Front/1
  ASMSignalCollector/1(ASMSignalBus) -> ASMSignalBus/1
  AirSuspensionSignals_In/1 -> SuspensionRear/5(AirSuspensionSignals_In), SuspensionFront/5(AirSuspensionSignals_In)
  SuspensionFront/3(v_Rel_WheelBody[FL,FR][x;y;z][m|s]) -> Mux5/1
  SuspensionFront/2(UnitVec_y_Wheel_CoorSys_V[FL,FR][x;y;z]) -> Mux15/1
  SuspensionRear/7(SuspensionKinematicRelations_Rear) -> SuspensionKinematicRelations_Rear/1
  SuspensionRear/2(UnitVec_y_Wheel_CoorSys_V[RL;RR][x;y;z][]) -> Mux15/2
  SuspensionFront/8(AirSuspensionSignals_Front) -> Terminator/1
  Mux1/1 -> gF_Susp[q1_Front;q2_Front;q1_Rear;q2_Rear][]/1
  Trq_Tire[FL;FR;RL;RR][x;y;z][Nm]/1 -> SuspensionRear/4(Trq_Tire[FL;FR;RL;RR][x;y;z][Nm]), SuspensionFront/4(Trq_Tire[FL;FR;RL;RR][x;y;z][Nm])
  Mux7/1 -> w_Rel_WheelBody[FL,FR,RL,RR][x;y;z][x;y;z][rad|s]/1
  SuspensionRear/3(v_Rel_WheelBody[RL;RR][x;y;z][m|s]) -> Mux5/2
  SuspensionFront/1("Pos_Wheel[FL,FR][x;y;z][m] ") -> Mux6/1
  F_Tire[FL;FR;RL;RR][x;y;z][N]/1 -> SuspensionRear/3(F_Tire[FL;FR;RL;RR][x;y;z][N]), SuspensionFront/3(F_Tire[FL;FR;RL;RR][x;y;z][N])
  SuspensionRear/1("Pos_Wheel[RL;RR][x;y;z][m] ") -> Mux6/2
  Mux15/1 -> UnitVec_y_Wheel_CoorSys_V[FL,FR,RL,RR][x;y;z]/1
  q_Wheel_dt[q1_Front;q2_Front;q1_Rear;q2_Rear][]/1 -> SuspensionRear/1(q_Wheel_dt[q1_Front;q2_Front;q1_Rear;q2_Rear][]), SuspensionFront/1(q_Wheel_dt[q1_Front;q2_Front;q1_Rear;q2_Rear][])

== system ASM_Traffic_new/VehicleDynamics/Plant/VehicleDynamics/Tire ==
  UnitVec_y_Wheel_CoorSys_V[FL,FR,RL,RR][x;y;z] : Inport
  RotationMatrix_V_to_E_T[3x3] : Inport  Port=2
  Pos_Wheels_CoorSys_E[FL,FR,RL,RR][x,y,z][m] : Inport  Port=3
  v_Abs_WheelBody_CoorSys_V[FL,FR,RL,RR][x;y;z][m|s] : Inport  Port=4
  w_Abs_Wheel_CoorSys_V[FL,FR,RL,RR][x,y,z][rad|s] : Inport  Port=5
  Sw_Tire_Parameter_Set[FL,FR,RL,RR][1|2|3|4] : Inport  Port=6
  Coef_Fric_Road[FL,FR,RL,RR][] : Inport  Port=7
  " Pos_z_CP_CoorSys_E[FL,FR,RL,RR][m]" : Inport  Port=8
  UnitVec_z_CP_CoorSys_E[FL,FR,RL,RR][x;y;z] : Inport  Port=9
  Reset[] : Inport  Port=10
  omega_Wheel[FL,FR,RL,RR][rad|s] : Inport  Port=11
  Sw_r_Tire[1:intern;2:extern] : Inport  Port=12
  r_Tire_extern[m] : Inport  Port=13
  ASMSignalCollector : Subsystem
  Bus Creator1 : BusCreator  Inputs=2
  Demux : Demux  Outputs=[1 1]
  Goto Tag Visibility : GotoTagVisibility  GotoTag=ASMBUS_VehicleDynamics_Tire_FL_ContactPoint
  Goto Tag Visibility1 : GotoTagVisibility  GotoTag=ASMBUS_VehicleDynamics_Tire_FL_Tire
  Goto Tag Visibility10 : GotoTagVisibility  GotoTag=ASMBUS_VehicleDynamics_Tire_RR_ForcesAndTorques
  Goto Tag Visibility16 : GotoTagVisibility  GotoTag=ASMBUS_VehicleDynamics_Tire_FR_ForcesAndTorques
  Goto Tag Visibility2 : GotoTagVisibility  GotoTag=ASMBUS_VehicleDynamics_Tire_FR_ContactPoint
  Goto Tag Visibility3 : GotoTagVisibility  GotoTag=ASMBUS_VehicleDynamics_Tire_FL_ForcesAndTorques
  Goto Tag Visibility4 : GotoTagVisibility  GotoTag=ASMBUS_VehicleDynamics_Tire_RL_ContactPoint
  Goto Tag Visibility5 : GotoTagVisibility  GotoTag=ASMBUS_VehicleDynamics_Tire_RL_Tire
  Goto Tag Visibility6 : GotoTagVisibility  GotoTag=ASMBUS_VehicleDynamics_Tire_FR_Tire
  Goto Tag Visibility7 : GotoTagVisibility  GotoTag=ASMBUS_VehicleDynamics_Tire_RL_ForcesAndTorques
  Goto Tag Visibility8 : GotoTagVisibility  GotoTag=ASMBUS_VehicleDynamics_Tire_RR_ContactPoint
  Goto Tag Visibility9 : GotoTagVisibility  GotoTag=ASMBUS_VehicleDynamics_Tire_RR_Tire
  Mux{1,3..5} (4 alike) : Mux
  Sat_TireParSet : Saturate  UpperLimit=4  LowerLimit=1
  Selector{1..2,14,32} (4 alike) : Selector  InputPortWidth=4  IndexOptions=Index vector (dialog)  Indices=[2]  OutputSizes=1
  Selector{3,9..10,31} (4 alike) : Selector  InputPortWidth=4  IndexOptions=Index vector (dialog)  Indices=[1]  OutputSizes=1
  Selector{7..8,11..13} (5 alike) : Selector  InputPortWidth=12  IndexOptions=Index vector (dialog)  Indices=[4 5 6]  OutputSizes=1
  Selector{15..16,22,33} (4 alike) : Selector  InputPortWidth=4  IndexOptions=Index vector (dialog)  Indices=[3]  OutputSizes=1
  Selector{17..21} (5 alike) : Selector  InputPortWidth=12  IndexOptions=Index vector (dialog)  Indices=[7 8 9]  OutputSizes=1
  Selector{23..25,34} (4 alike) : Selector  InputPortWidth=4  IndexOptions=Index vector (dialog)  Indices=[4]  OutputSizes=1
  Selector{26..30} (5 alike) : Selector  InputPortWidth=12  IndexOptions=Index vector (dialog)  Indices=[10 11 12]  OutputSizes=1
  Selector{4..6,37..38} (5 alike) : Selector  InputPortWidth=12  IndexOptions=Index vector (dialog)  Indices=[1 2 3]  OutputSizes=1
  TIRE_MODE : ASM_VehicleDynamics_lib/VehicleDynamics/Tire/Base/TIRE_MODE  Tag=ASM_SUBCOMPONENT  ModeLeft=MDL.VehicleDynamics.Tire.ModeLeft  ModeRight=MDL.VehicleDynamics.Tire.ModeRight  ASMProperties=struct('Name','TIRE_MODE','Version','1.0','Library','ASM_VehicleDynamics_lib')  ASMInstanceName=tire_mode  ASMInstanceID=1
  Tire_FL : Subsystem
  Tire_FR : Subsystem
  Tire_RL : Subsystem
  Tire_RR : Subsystem
  p[Pa] : Constant  Value=220000
  ASMSignalBus : Outport  VectorParamsAs1DForOutWhenUnconnected=off
  F_Tire_CoorSys_V[FL,FR,RL,RR][x;y;z][N] : Outport  Port=2  VectorParamsAs1DForOutWhenUnconnected=off
  Trq_Tire_CoorSys_V[FL,FR,RL,RR][x;y;z][Nm] : Outport  Port=3  VectorParamsAs1DForOutWhenUnconnected=off
  Stiffness_z_Tire[FL,FR,RL,RR][N|m] : Outport  Port=4  VectorParamsAs1DForOutWhenUnconnected=off
  Trq_Tire_Wheel[FL,FR,RL,RR][Nm] : Outport  Port=5  VectorParamsAs1DForOutWhenUnconnected=off
  wires:
  ASMSignalCollector/1(ASMSignalBus) -> ASMSignalBus/1
  Mux4/1 -> F_Tire_CoorSys_V[FL,FR,RL,RR][x;y;z][N]/1
  Mux1/1 -> Trq_Tire_CoorSys_V[FL,FR,RL,RR][x;y;z][Nm]/1
  Selector10/1 -> Tire_FL/9(omega_Wheel[rad|s])
  omega_Wheel[FL,FR,RL,RR][rad|s]/1 -> Selector24/1, Selector22/1, Selector1/1, Selector10/1
  Selector37/1 -> Tire_FL/8(UnitVec_y_Wheel_CoorSys_V[x;y;z])
  UnitVec_y_Wheel_CoorSys_V[FL,FR,RL,RR][x;y;z]/1 -> Selector30/1, Selector21/1, Selector7/1, Selector37/1
  RotationMatrix_V_to_E_T[3x3]/1 -> Tire_RR/7(RotationMatrix_V_to_E_T[3x3]), Tire_RL/7(RotationMatrix_V_to_E_T[3x3]), Tire_FR/7(RotationMatrix_V_to_E_T[3x3]), Tire_FL/7(RotationMatrix_V_to_E_T[3x3])
  UnitVec_z_CP_CoorSys_E[FL,FR,RL,RR][x;y;z]/1 -> Selector26/1, Selector17/1, Selector11/1, Selector4/1
  " Pos_z_CP_CoorSys_E[FL,FR,RL,RR][m]"/1 -> Selector25/1, Selector16/1, Selector2/1, Selector3/1
  Selector3/1 -> Tire_FL/2(" Pos_z_CP_CoorSys_E[m]")
  Selector9/1 -> Tire_FL/1(Coeff_Fric_Road[])
  Coef_Fric_Road[FL,FR,RL,RR][]/1 -> Selector23/1, Selector15/1, Selector14/1, Selector9/1
  Selector4/1 -> Tire_FL/3(UnitVec_z_CP_CoorSys_E[x;y;z])
  Pos_Wheels_CoorSys_E[FL,FR,RL,RR][x,y,z][m]/1 -> Selector27/1, Selector18/1, Selector12/1, Selector5/1
  Selector5/1 -> Tire_FL/4(Pos_Wheels_CoorSys_E[x;y;z][m])
  v_Abs_WheelBody_CoorSys_V[FL,FR,RL,RR][x;y;z][m|s]/1 -> Selector28/1, Selector19/1, Selector8/1, Selector6/1
  Selector6/1 -> Tire_FL/5(v_Abs_WheelBody_CoorSys_V[x;y;z][m|s])
  w_Abs_Wheel_CoorSys_V[FL,FR,RL,RR][x,y,z][rad|s]/1 -> Selector29/1, Selector20/1, Selector13/1, Selector38/1
  Selector38/1 -> Tire_FL/6(w_Abs_Wheel_CoorSys_V[x;y;z][rad|s])
  Selector14/1 -> Tire_FR/1(Coeff_Fric_Road[])
  Selector2/1 -> Tire_FR/2(" Pos_z_CP_CoorSys_E[m]")
  Selector11/1 -> Tire_FR/3(UnitVec_z_CP_CoorSys_E[x;y;z])
  Selector12/1 -> Tire_FR/4(Pos_Wheels_CoorSys_E[x;y;z][m])
  Selector8/1 -> Tire_FR/5(v_Abs_WheelBody_CoorSys_V[x;y;z][m|s])
  Selector13/1 -> Tire_FR/6(w_Abs_Wheel_CoorSys_V[x;y;z][rad|s])
  Selector7/1 -> Tire_FR/8(UnitVec_y_Wheel_CoorSys_V[x;y;z])
  Selector1/1 -> Tire_FR/9(omega_Wheel[rad|s])
  Selector15/1 -> Tire_RL/1(Coeff_Fric_Road[])
  Selector16/1 -> Tire_RL/2(" Pos_z_CP_CoorSys_E[m]")
  Selector17/1 -> Tire_RL/3(UnitVec_z_CP_CoorSys_E[x;y;z])
  Selector18/1 -> Tire_RL/4(Pos_Wheels_CoorSys_E[x;y;z][m])
  Selector19/1 -> Tire_RL/5(v_Abs_WheelBody_CoorSys_V[x;y;z][m|s])
  Selector20/1 -> Tire_RL/6(w_Abs_Wheel_CoorSys_V[x;y;z][rad|s])
  Selector21/1 -> Tire_RL/8(UnitVec_y_Wheel_CoorSys_V[x;y;z])
  Selector22/1 -> Tire_RL/9(omega_Wheel[rad|s])
  Tire_FL/1(F_Tire[x;y;z][N]) -> Mux4/1
  Tire_FR/1(F_Tire[x;y;z][N]) -> Mux4/2
  Tire_RL/1(F_Tire[x;y;z][N]) -> Mux4/3
  Tire_RR/1(F_Tire[x;y;z][N]) -> Mux4/4
  Tire_FL/2(Trq_Tire[x;y;z][Nm]) -> Mux1/1
  Tire_FR/2(Trq_Tire[x;y;z][Nm]) -> Mux1/2
  Tire_RL/2(Trq_Tire[x;y;z][Nm]) -> Mux1/3
  Tire_RR/2(Trq_Tire[x;y;z][Nm]) -> Mux1/4
  Mux3/1 -> Trq_Tire_Wheel[FL,FR,RL,RR][Nm]/1
  Tire_FL/3(Trq_Tire_Wheel[Nm]) -> Mux3/1
  Tire_FR/3(Trq_Tire_Wheel[Nm]) -> Mux3/2
  Tire_RL/3(Trq_Tire_Wheel[Nm]) -> Mux3/3
  Tire_RR/3(Trq_Tire_Wheel[Nm]) -> Mux3/4
  Sw_Tire_Parameter_Set[FL,FR,RL,RR][1|2|3|4]/1 -> Sat_TireParSet/1
  Selector31/1 -> Tire_FL/10(Sw_Tire_Parameter_Set[1|2|3|4])
  Selector32/1 -> Tire_FR/10(Sw_Tire_Parameter_Set[1|2|3|4])
  Selector33/1 -> Tire_RL/10(Sw_Tire_Parameter_Set[1|2|3|4])
  Selector34/1 -> Tire_RR/10(Sw_Tire_Parameter_Set[1|2|3|4])
  Selector30/1 -> Tire_RR/8(UnitVec_y_Wheel_CoorSys_V[x;y;z])
  Selector24/1 -> Tire_RR/9(omega_Wheel[rad|s])
  Selector29/1 -> Tire_RR/6(w_Abs_Wheel_CoorSys_V[x;y;z][rad|s])
  Selector28/1 -> Tire_RR/5(v_Abs_WheelBody_CoorSys_V[x;y;z][m|s])
  Selector27/1 -> Tire_RR/4(Pos_Wheels_CoorSys_E[x;y;z][m])
  Selector26/1 -> Tire_RR/3(UnitVec_z_CP_CoorSys_E[x;y;z])
  Selector25/1 -> Tire_RR/2(" Pos_z_CP_CoorSys_E[m]")
  Selector23/1 -> Tire_RR/1(Coeff_Fric_Road[])
  Tire_FL/4(Stiffness_z_Tire[N|m]) -> Mux5/1
  Tire_FR/4(Stiffness_z_Tire[N|m]) -> Mux5/2
  Tire_RL/4(Stiffness_z_Tire[N|m]) -> Mux5/3
  Tire_RR/4(Stiffness_z_Tire[N|m]) -> Mux5/4
  Mux5/1 -> Stiffness_z_Tire[FL,FR,RL,RR][N|m]/1
  Reset[]/1 -> Tire_RR/11(Reset[]), Tire_RL/11(Reset[]), Tire_FR/11(Reset[]), Tire_FL/11(Reset[])
  Sat_TireParSet/1 -> Selector34/1, Selector33/1, Selector32/1, Selector31/1
  Demux/1 -> Tire_RL/12(Mode[1Normal|2Mirror|3Symmetric]), Tire_FL/12(Mode[1Normal|2Mirror|3Symmetric])
  p[Pa]/1 -> Tire_RR/13(p[Pa]), Tire_RL/13(p[Pa]), Tire_FR/13(p[Pa]), Tire_FL/13(p[Pa])
  Demux/2 -> Tire_RR/12(Mode[1Normal|2Mirror|3Symmetric]), Tire_FR/12(Mode[1Normal|2Mirror|3Symmetric])
  TIRE_MODE/1 -> Demux/1
  Sw_r_Tire[1:intern;2:extern]/1 -> Bus Creator1/1
  r_Tire_extern[m]/1 -> Bus Creator1/2
  Bus Creator1/1 -> Tire_RR/14(Tire_Switches), Tire_RL/14(Tire_Switches), Tire_FR/14(Tire_Switches), Tire_FL/14(Tire_Switches)
